simulink model "DCHR_Dispatch_Stateflow_v32"  (R2026a)
settings: Solver=FixedStepDiscrete  StopTime=dchr_stop_v32  FixedStep=dchr_dt_v32
model workspace (MAT data in the model file):
  dchr_E0_v32 = 9
  dchr_dt_v32 = 1
  dchr_h_v32 = [8 0.45 1.2 8 0.08 0 4 0 0]
  dchr_input_v32 = [0  6  35  75  0  45; 1  0  35  75  5  45]
  dchr_p_v32 = [1 10 3 4 0.9 0.8 0.1 5 0.2 20 2]
  dchr_stop_v32 = 1
settings Model: Creator=Lysda  LastModifiedBy=Lysda

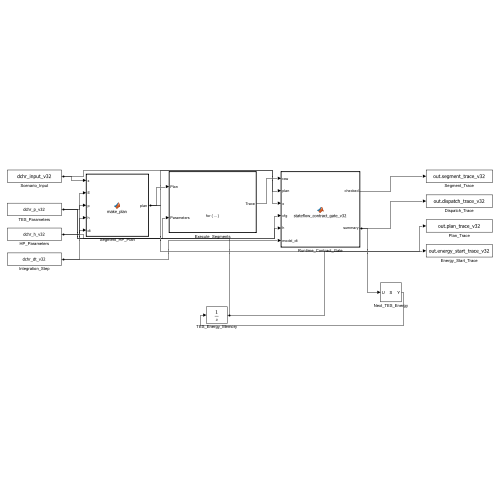
[thumbnail: Simulink's stored preview of the top-level diagram]
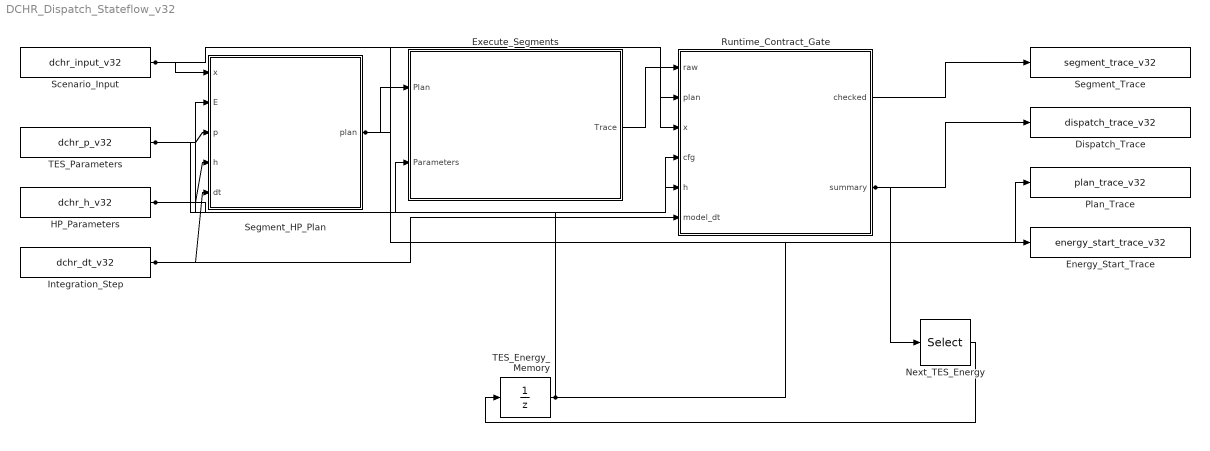
== system DCHR_Dispatch_Stateflow_v32 ==
  Dispatch_Trace : ToWorkspace  VariableName=dispatch_trace_v32  SaveFormat=Timeseries  SampleTime=-1
  Energy_Start_Trace : ToWorkspace  VariableName=energy_start_trace_v32  SaveFormat=Timeseries  SampleTime=-1
  Execute_Segments : Subsystem  TreatAsAtomicUnit=on
  HP_Parameters : Constant  Value=dchr_h_v32
  Integration_Step : Constant  Value=dchr_dt_v32
  Next_TES_Energy : Selector  InputPortWidth=25  IndexOptions=Index vector (dialog)  Indices=8  OutputSizes=1
  Plan_Trace : ToWorkspace  VariableName=plan_trace_v32  SaveFormat=Timeseries  SampleTime=-1
  Runtime_Contract_Gate : MATLAB Function  TreatAsAtomicUnit=on
  Scenario_Input : FromWorkspace  VariableName=dchr_input_v32  SampleTime=dchr_dt_v32  Interpolate=off  OutputAfterFinalValue=Holding final value
  Segment_HP_Plan : MATLAB Function  TreatAsAtomicUnit=on
  Segment_Trace : ToWorkspace  VariableName=segment_trace_v32  SaveFormat=Timeseries  SampleTime=-1
  TES_Energy_Memory : UnitDelay  InitialCondition=dchr_E0_v32  SampleTime=dchr_dt_v32
  TES_Parameters : Constant  Value=dchr_p_v32
  wires:
  Scenario_Input/1 -> Segment_HP_Plan/1(x), Runtime_Contract_Gate/3(x)
  TES_Energy_Memory/1 -> Segment_HP_Plan/2(E), Energy_Start_Trace/1
  TES_Parameters/1 -> Segment_HP_Plan/3(p), Execute_Segments/2(Parameters), Runtime_Contract_Gate/4(cfg)
  HP_Parameters/1 -> Segment_HP_Plan/4(h), Runtime_Contract_Gate/5(h)
  Integration_Step/1 -> Segment_HP_Plan/5(dt), Runtime_Contract_Gate/6(model_dt)
  Segment_HP_Plan/1(plan) -> Execute_Segments/1(Plan), Runtime_Contract_Gate/2(plan), Plan_Trace/1
  Execute_Segments/1(Trace) -> Runtime_Contract_Gate/1(raw)
  Runtime_Contract_Gate/1(checked) -> Segment_Trace/1
  Runtime_Contract_Gate/2(summary) -> Dispatch_Trace/1, Next_TES_Energy/1
  Next_TES_Energy/1 -> TES_Energy_Memory/1

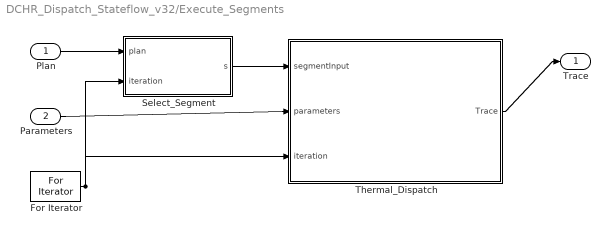
== system DCHR_Dispatch_Stateflow_v32/Execute_Segments ==
  Plan : Inport
  Parameters : Inport  Port=2
  For Iterator : ForIterator  IterationLimit=2
  Select_Segment : MATLAB Function  TreatAsAtomicUnit=on
  Thermal_Dispatch : Stateflow chart  TreatAsAtomicUnit=on
  Trace : Outport
  wires:
  Plan/1 -> Select_Segment/1(plan)
  For Iterator/1 -> Select_Segment/2(iteration), Thermal_Dispatch/3(iteration)
  Select_Segment/1(s) -> Thermal_Dispatch/1(segmentInput)
  Parameters/1 -> Thermal_Dispatch/2(parameters)
  Thermal_Dispatch/1(Trace) -> Trace/1

== matlab function DCHR_Dispatch_Stateflow_v32/Runtime_Contract_Gate ==
  data: raw input; checked output; plan input; x input; cfg input; h input; model_dt input; summary output
function [checked,summary]=stateflow_contract_gate_v32(raw,plan,x,cfg,h,model_dt)
%#codegen
% Per-segment independent ODE/HP/service laws, then integrate powers.
dt=cfg(1);cap=cfg(2);rate=cfg(7);ec=cfg(5);ed=cfg(6);
assert(all(isfinite(cfg)) && dt==model_dt && dt>0,'Invalid model interval.');
assert(all(isfinite(x)) && all(isfinite(h)),'Invalid host inputs.');
energy=zeros(9,1);loss=zeros(3,1);highest=0;
for k=1:2
    z=raw((k-1)*25+(1:25));s=plan(:,k);span=z(2);
    finite=z;finite(15)=0;
    assert(all(isfinite(finite)) && all(isfinite(s([1:7 9:14]))),'Nonfinite segment.');
    tol=1e-9*max(1,cap+(z(11)+cfg(11))*dt);ptol=tol/max(dt,eps);
    assert(span>=0 && span==s(1) && z(3)==s(14) && abs(z(4)-s(2))<=tol,'Segment schedule mismatch.');
    assert(z(1)==floor(z(1)) && z(1)>=0 && z(1)<=5,'Undefined segment state.');
    assert(min(z(4:5))>=-tol && max(z(4:5))<=cap+tol,'TES bounds failure.');
    assert(all(z(6:14)>=-ptol) && all(z(16:20)>=-tol),'Negative flows/losses.');
    assert(z(7)<=cfg(3)+ptol && z(8)<=cfg(4)+ptol && z(9)<=cfg(11)+ptol && z(7)*z(8)==0,'Instantaneous port limits.');
    if span>0
        P=ec*z(7)-z(8)/ed;r=exp(-rate*span);phi=span;
        if rate>0 && rate*span>0,phi=-expm1(-rate*span)/rate;end
        assert(abs(z(5)-(z(4)*r+P*phi))<=tol,'Segment ODE failure.');
        assert(z(8)==0 || min(z(4:5))>=cfg(8)-tol,'Discharge crosses cutoff.');
        assert(abs(z(17)-(z(4)+P*span-z(5)))<=tol && ...
            abs(z(18)-(1-ec)*z(7)*span)<=tol && abs(z(19)-(1/ed-1)*z(8)*span)<=tol,'Segment losses failure.');
        assert(abs(z(11)-z(12)-z(13))*span<=tol && abs(z(11)-z(6)-z(7))*span<=tol,'HP first law/allocation failure.');
        assert(abs(x(4)-z(6)-z(8)-z(9)-z(10))*span<=tol && ...
            abs(z(20)-z(6)-z(8)-z(9))*span<=tol,'Segment service closure.');
        expected=0;
        if z(10)>0,expected=5;elseif z(9)>0,expected=4;elseif z(8)>0,expected=3;
        elseif z(7)>0,expected=2;elseif z(6)>0,expected=1;end
        assert(z(1)==expected,'State does not authorize actual segment flows.');
        assert(abs(x(1)-z(13)-z(16))<=ptol && z(11)<=h(1)+ptol && z(11)<=z(14)+ptol,'Source/request/capacity limit.');
        if z(11)>0
            carnot=(x(3)+273.15)/(x(3)-x(2));
            nominal=h(2)*carnot;if h(6)==1,nominal=h(7)+h(8)*(x(3)-x(2))+h(9)*(x(3)-x(2))^2;end
            expectedCOP=min(h(4),nominal)*(1-h(5)+h(5)*z(11)/h(1));
            assert(isfinite(z(15)) && z(15)>=h(3)-ptol && z(15)<=carnot+ptol && z(25)==1 && ...
                abs(z(15)-expectedCOP)<=ptol && abs(z(12)*z(15)-z(11))<=ptol,'Segment COP failure.');
        else,assert(isnan(z(15)) && z(25)==0,'Off HP convention.');end
        highest=max(highest,z(1));
    else
        assert(z(1)==0 && all(z(6:14)==0) && all(z(17:21)==0) && z(5)==z(4),'Zero-span segment has service.');
    end
    assert(abs(z(22)-(cfg(10)+z(4)/cfg(9)))<=tol/cfg(9) && ...
        abs(z(23)-(cfg(10)+z(5)/cfg(9)))<=tol/cfg(9),'Segment temperature mismatch.');
    residual=z(4)+(z(13)+z(12)+z(9)-z(20))*span-z(5)-sum(z(17:19));
    assert(abs(residual)<=tol && abs(z(21)-residual)<=tol,'Segment system balance failure.');
    assert(z(24)==s(13) && ismember(z(24),[0 1 2]),'Invalid event kind.');
    energy=energy+[z(6:14)]*span;loss=loss+z(17:19);
end
first=raw(1:25);last=raw(26:50);
tol=1e-9*max(1,cap+(energy(6)+cfg(11)*dt));
assert(abs(first(2)+last(2)-dt)<=tol && first(3)==0 && abs(last(3)-first(2))<=tol,'Interval partition failure.');
assert(abs(first(5)-last(4))<=tol,'Event handoff energy mismatch.');
if last(2)>0 && first(24)==1,assert(abs(first(5)-cap)<=tol && last(8)==0,'Capacity boundary failure.');end
if last(2)>0 && first(24)==2,assert(abs(first(5)-cfg(8))<=tol && last(8)==0,'Cutoff boundary failure.');end
supplied=(energy(1)+energy(3)+energy(4))/dt;
residual=first(4)+energy(7)+energy(8)+energy(4)-supplied*dt-last(5)-sum(loss);
assert(abs(residual)<=tol,'Integrated first law failure.');
cop=NaN;if energy(7)>0,cop=energy(6)/energy(7);end
summary=[highest;energy(1:5)/dt;first(4)*exp(-rate*dt);last(5);loss;supplied;residual; ...
    first(22);last(23);max(0,first(4)-cfg(8));max(0,last(5)-cfg(8)); ...
    x(4);energy(6:9)/dt;cop;double(energy(6)>0);x(1)-energy(8)/dt];
checked=raw;
end

== matlab function DCHR_Dispatch_Stateflow_v32/Execute_Segments/Select_Segment ==
  data: plan input; s output; iteration input
function s=pick(plan,iteration)
%#codegen
s=plan(:,iteration);
end

== matlab function DCHR_Dispatch_Stateflow_v32/Segment_HP_Plan ==
  data: x input; plan output; E input; p input; h input; dt input
function plan=make_plan(x,E,p,h,dt)
%#codegen
coder.extrinsic('dchr_segment_plan_v32');
plan=zeros(14,2);
plan=dchr_segment_plan_v32(x,E,p,h,dt);
end

== stateflow chart DCHR_Dispatch_Stateflow_v32/Execute_Segments/Thermal_Dispatch ==
  settings: description=Release 0.32: two ordered analytic intra-interval segments; actual guarded state execution each iteration. Offsets are physical event times; Simulink clock stays at macro sample start. Normal-mode host HP.
  state IDLE
    en,du:
    if iteration==1
    Trace=zeros(50,1);
    end
    segmentOutput=stateflow_allocate_v32(0,segmentInput,parameters);
    Trace=stateflow_collect_v32(Trace,segmentOutput,iteration);
  state HEAT_RECOVERY
    en,du:
    if iteration==1
    Trace=zeros(50,1);
    end
    segmentOutput=stateflow_allocate_v32(1,segmentInput,parameters);
    Trace=stateflow_collect_v32(Trace,segmentOutput,iteration);
  state STORAGE_CHARGE
    en,du:
    if iteration==1
    Trace=zeros(50,1);
    end
    segmentOutput=stateflow_allocate_v32(2,segmentInput,parameters);
    Trace=stateflow_collect_v32(Trace,segmentOutput,iteration);
  state STORAGE_DISCHARGE
    en,du:
    if iteration==1
    Trace=zeros(50,1);
    end
    segmentOutput=stateflow_allocate_v32(3,segmentInput,parameters);
    Trace=stateflow_collect_v32(Trace,segmentOutput,iteration);
  state BACKUP
    en,du:
    if iteration==1
    Trace=zeros(50,1);
    end
    segmentOutput=stateflow_allocate_v32(4,segmentInput,parameters);
    Trace=stateflow_collect_v32(Trace,segmentOutput,iteration);
  state UNMET_DEMAND
    en,du:
    if iteration==1
    Trace=zeros(50,1);
    end
    segmentOutput=stateflow_allocate_v32(5,segmentInput,parameters);
    Trace=stateflow_collect_v32(Trace,segmentOutput,iteration);
  (junction 26) -> STORAGE_CHARGE [order 3] : [stateflow_choose_mode_v32(segmentInput,parameters)==2]
  (junction 26) -> HEAT_RECOVERY [order 2] : [stateflow_choose_mode_v32(segmentInput,parameters)==1]
  (default) -> (junction 26)
  (junction 26) -> IDLE [order 1] : [stateflow_choose_mode_v32(segmentInput,parameters)==0]
  (junction 26) -> UNMET_DEMAND [order 6] : [stateflow_choose_mode_v32(segmentInput,parameters)==5]
  (junction 26) -> STORAGE_DISCHARGE [order 4] : [stateflow_choose_mode_v32(segmentInput,parameters)==3]
  (junction 26) -> BACKUP [order 5] : [stateflow_choose_mode_v32(segmentInput,parameters)==4]
  STORAGE_CHARGE -> STORAGE_DISCHARGE [order 3] : [stateflow_choose_mode_v32(segmentInput,parameters)==3]
  HEAT_RECOVERY -> STORAGE_DISCHARGE [order 3] : [stateflow_choose_mode_v32(segmentInput,parameters)==3]
  STORAGE_CHARGE -> BACKUP [order 4] : [stateflow_choose_mode_v32(segmentInput,parameters)==4]
  UNMET_DEMAND -> IDLE [order 1] : [stateflow_choose_mode_v32(segmentInput,parameters)==0]
  STORAGE_DISCHARGE -> IDLE [order 1] : [stateflow_choose_mode_v32(segmentInput,parameters)==0]
  STORAGE_CHARGE -> IDLE [order 1] : [stateflow_choose_mode_v32(segmentInput,parameters)==0]
  BACKUP -> IDLE [order 1] : [stateflow_choose_mode_v32(segmentInput,parameters)==0]
  HEAT_RECOVERY -> IDLE [order 1] : [stateflow_choose_mode_v32(segmentInput,parameters)==0]
  STORAGE_DISCHARGE -> HEAT_RECOVERY [order 2] : [stateflow_choose_mode_v32(segmentInput,parameters)==1]
  STORAGE_DISCHARGE -> STORAGE_CHARGE [order 3] : [stateflow_choose_mode_v32(segmentInput,parameters)==2]
  BACKUP -> HEAT_RECOVERY [order 2] : [stateflow_choose_mode_v32(segmentInput,parameters)==1]
  UNMET_DEMAND -> HEAT_RECOVERY [order 2] : [stateflow_choose_mode_v32(segmentInput,parameters)==1]
  STORAGE_CHARGE -> HEAT_RECOVERY [order 2] : [stateflow_choose_mode_v32(segmentInput,parameters)==1]
  IDLE -> HEAT_RECOVERY [order 1] : [stateflow_choose_mode_v32(segmentInput,parameters)==1]
  IDLE -> STORAGE_CHARGE [order 2] : [stateflow_choose_mode_v32(segmentInput,parameters)==2]
  BACKUP -> STORAGE_CHARGE [order 3] : [stateflow_choose_mode_v32(segmentInput,parameters)==2]
  UNMET_DEMAND -> STORAGE_CHARGE [order 3] : [stateflow_choose_mode_v32(segmentInput,parameters)==2]
  HEAT_RECOVERY -> STORAGE_CHARGE [order 2] : [stateflow_choose_mode_v32(segmentInput,parameters)==2]
  IDLE -> STORAGE_DISCHARGE [order 3] : [stateflow_choose_mode_v32(segmentInput,parameters)==3]
  HEAT_RECOVERY -> BACKUP [order 4] : [stateflow_choose_mode_v32(segmentInput,parameters)==4]
  STORAGE_CHARGE -> UNMET_DEMAND [order 5] : [stateflow_choose_mode_v32(segmentInput,parameters)==5]
  IDLE -> BACKUP [order 4] : [stateflow_choose_mode_v32(segmentInput,parameters)==4]
  IDLE -> UNMET_DEMAND [order 5] : [stateflow_choose_mode_v32(segmentInput,parameters)==5]
  HEAT_RECOVERY -> UNMET_DEMAND [order 5] : [stateflow_choose_mode_v32(segmentInput,parameters)==5]
  UNMET_DEMAND -> STORAGE_DISCHARGE [order 4] : [stateflow_choose_mode_v32(segmentInput,parameters)==3]
  BACKUP -> STORAGE_DISCHARGE [order 4] : [stateflow_choose_mode_v32(segmentInput,parameters)==3]
  UNMET_DEMAND -> BACKUP [order 5] : [stateflow_choose_mode_v32(segmentInput,parameters)==4]
  STORAGE_DISCHARGE -> BACKUP [order 4] : [stateflow_choose_mode_v32(segmentInput,parameters)==4]
  STORAGE_DISCHARGE -> UNMET_DEMAND [order 5] : [stateflow_choose_mode_v32(segmentInput,parameters)==5]
  BACKUP -> UNMET_DEMAND [order 5] : [stateflow_choose_mode_v32(segmentInput,parameters)==5]
  data: seg function_input; cfg function_input; mode function_output; mode function_input; seg function_input; cfg function_input; z function_output; previous function_input; z function_input; index function_input; packed function_output; segmentInput input double size=[14 1]; parameters input double size=[1 11]; iteration input int32 size=1; Trace output double size=[50 1]; segmentOutput local double size=[25 1]
  function mode=stateflow_choose_mode_v32(seg,cfg):
    | function mode=stateflow_choose_mode_v32(seg,cfg)
    | %#codegen
    | % Guard each positive-duration segment using instantaneous service deficit.
    | direct=min(seg(3),seg(4));remaining=max(0,seg(3)-direct-seg(12));
    | mode=0;
    | if seg(1)==0,return;end
    | if remaining>cfg(11),mode=5;
    | elseif remaining>0,mode=4;
    | elseif seg(12)>0,mode=3;
    | elseif seg(11)>0,mode=2;
    | elseif direct>0,mode=1;
    | end
    | end
  function z=stateflow_allocate_v32(mode,seg,cfg):
    | function z=stateflow_allocate_v32(mode,seg,cfg)
    | %#codegen
    | % Actual Stateflow state authorizes instantaneous TES and finite boiler ports.
    | span=seg(1);A=seg(2);direct=0;qc=0;qd=0;gas=0;unmet=0;
    | if span>0
    |     if mode>=1,direct=min(seg(3),seg(4));end
    |     if mode==2,qc=seg(11);end
    |     if mode>=3,qd=seg(12);end
    |     if mode>=4,gas=min(cfg(11),max(0,seg(3)-direct-qd));end
    |     if mode==5,unmet=max(0,seg(3)-direct-qd-gas);end
    | end
    | P=cfg(5)*qc-qd/cfg(6);rate=cfg(7);x=rate*span;
    | r=exp(-x);f=-expm1(-x);phi=span;beta=0;
    | if rate>0 && x>0
    |     phi=f/rate;
    |     if x<1e-4,beta=span*x*(.5-x*(1/6-x*(1/24-x*(1/120-x/720))));
    |     else,beta=span-phi;end
    | end
    | endpoint=A*r+P*phi;standing=A*f+P*beta;
    | % Roundoff correction only; reject any material bound crossing before clipping.
    | roundoff=64*eps(max(1,cfg(2)));
    | assert(endpoint>=-roundoff && endpoint<=cfg(2)+roundoff,'TES segment crosses physical capacity.');
    | endpoint=min(cfg(2),max(0,endpoint));
    | if qd>0 && seg(13)==2 && abs(endpoint-cfg(8))<=roundoff,endpoint=cfg(8);end
    | lc=(1-cfg(5))*qc*span;ld=(1/cfg(6)-1)*qd*span;
    | supplied=direct+qd+gas;
    | residual=(seg(6)+seg(5)+gas)*span+A-supplied*span-endpoint-standing-lc-ld;
    | z=[mode;span;seg(14);A;endpoint;direct;qc;qd;gas;unmet;seg(4:8);seg(10); ...
    |     standing;lc;ld;supplied;residual;cfg(10)+A/cfg(9);cfg(10)+endpoint/cfg(9);seg(13);seg(9)];
    | end
  function packed=stateflow_collect_v32(previous,z,index):
    | function packed=stateflow_collect_v32(previous,z,index)
    | %#codegen
    | % Two calls per macro sample: preserve separate executed segment outputs.
    | assert(index==1 || index==2,'Unexpected segment iteration.');
    | packed=previous;
    | if index==1,packed=zeros(50,1);end
    | if index==1,packed(1:25)=z;else,packed(26:50)=z;end
    | end
